simulink model "main_simulation"  (R2023a)
settings: Solver=VariableStepAuto  StartTime=0.0  StopTime=10.0  RelTol=1e-3
values from neighbouring files (symbols this model uses):
  A = [0 1 0 0 0 0 0 0 0 0 0 0 ... (first row only)    [main.m]
  a1 = (Iy - Iz) / Ix    (= 0.245886595932)    [main.m]
  a2 = (Iz - Ix) / Iy    (= -0.245886595932)    [main.m]
  a3 = (Ix - Iy) / Iz    (= 0)    [main.m]
  B = [0 0 0 0 ... (first row only)    [main.m]
  b1 = l / Ix    (= 2894.59486758)    [main.m]
  b2 = l / Iy    (= 2894.59486758)    [main.m]
  b3 = l / Iz    (= 3838.40792639)    [main.m]
  C = [1 0 0 0 0 0 0 0 0 0 0 0 ... (first row only)    [main.m]
  C1 = [0 0 0 0 1 0 0 0 0 0 0 0 ... (first row only)    [main.m]
  D = 0    [main.m]
  F_r = diag([-2,-2,-3,-3,-4,-4,-5,-5])    [main.m]
  g = 9.8    [main.m]
  inv_G_CL_0 = inv(G_CL_0)    [main.m]
  k = place(A, B, [-6.8-7.2i, -6.8+7.2i, -35, -35, -36, -36, -37, -37, -38, -38, -39, -39])    [main.m]
  K_d_LQR = K_LQR(:, 1:12)    [main.m]
  K_place = place(A,B,poles)    [main.m]
  K_q_LQR = K_LQR(:, 13:16)    [main.m]
  L = K'    [main.m]
  L_r = [rand(8,4)]    [main.m]
  m = 0.506    [main.m]
  Q_1 = inv_c_T(:,1:q)    [main.m]
  Q_2 = inv_c_T(:,q+1:n)    [main.m]
  T = lyap(F_r, -A, L_r * C1)    [main.m]
libraries: simulink x2, sim3dlib x1, uavsim3dlib x1
settings Model: Creator=Sheyda  LastModifiedBy=Sheyda

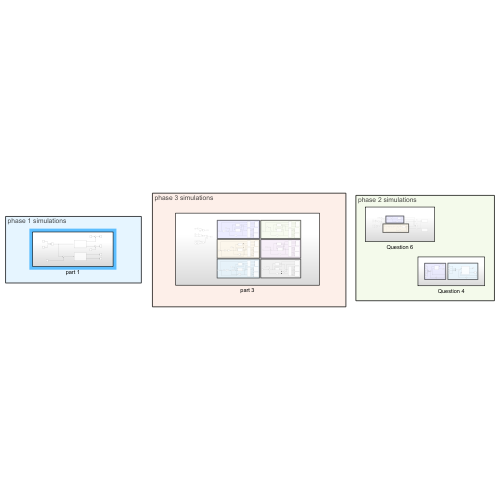
[thumbnail: Simulink's stored preview of the top-level diagram]
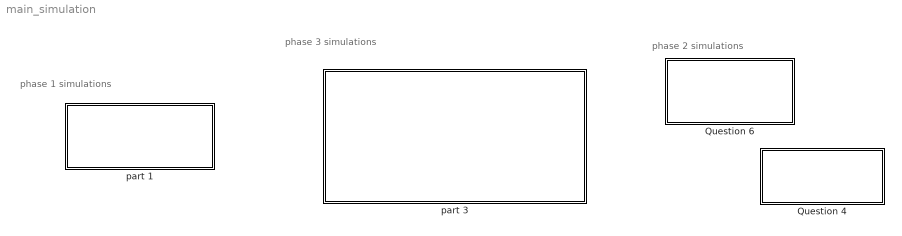
== system main_simulation ==
  note: phase 1 simulations
  note: phase 2 simulations
  note: phase 3 simulations
  Question 4 : Subsystem
  Question 6 : Subsystem
  part 1 : Subsystem
  part 3 : Subsystem

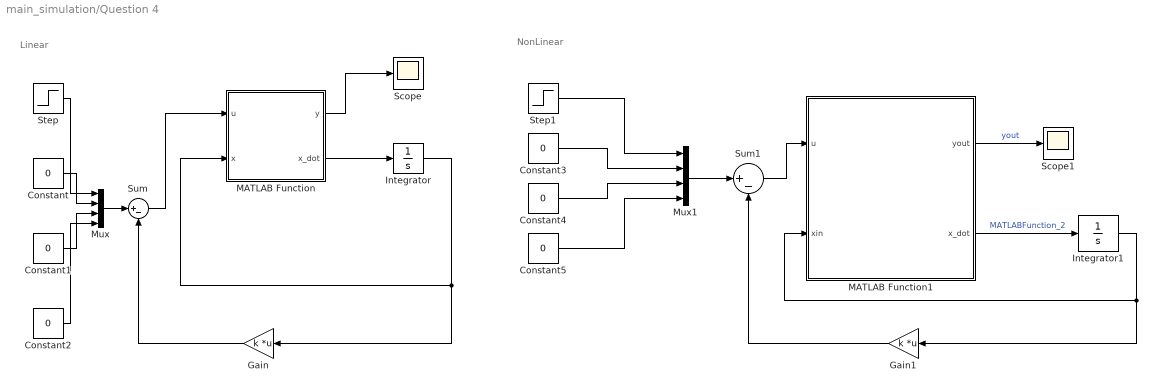
== system main_simulation/Question 4 ==
  note: Linear
  note: NonLinear
  Constant{,1..5} (6 alike) : Constant  Value=0
  Gain : Gain  Gain=k  Multiplication=Matrix(K*u)
  Gain1 : Gain  Gain=k  Multiplication=Matrix(K*u)
  Integrator : Integrator  InitialCondition=[0,0,0,0,0,0,0,0,0,0,0,0]'
  Integrator1 : Integrator  InitialCondition=[0,0,0,0,0,0,0,0,0,0,0,0]'
  MATLAB Function : MATLAB Function  TreatAsAtomicUnit=on
  MATLAB Function1 : MATLAB Function  TreatAsAtomicUnit=on
  Mux : Mux
  Mux1 : Mux
  Scope : Scope
  Scope1 : Scope
  Step : Step  SampleTime=0
  Step1 : Step  SampleTime=0
  Sum : Sum  Inputs=|+-
  Sum1 : Sum  Inputs=|+-
  wires:
  Constant/1 -> Mux/2
  Constant2/1 -> Mux/4
  Constant1/1 -> Mux/3
  Sum/1 -> MATLAB Function/1(u)
  Mux/1 -> Sum/1
  MATLAB Function/2(x_dot) -> Integrator/1
  Gain/1 -> Sum/2
  Integrator/1 -> MATLAB Function/2(x), Gain/1
  Step/1 -> Mux/1
  MATLAB Function/1(y) -> Scope/1
  Constant4/1 -> Mux1/3
  Step1/1 -> Mux1/1
  Constant5/1 -> Mux1/4
  Constant3/1 -> Mux1/2
  Sum1/1 -> MATLAB Function1/1(u)
  MATLAB Function1/2(x_dot) -> Integrator1/1  "MATLABFunction_2"
  MATLAB Function1/1(yout) -> Scope1/1  "yout"
  Mux1/1 -> Sum1/1
  Gain1/1 -> Sum1/2
  Integrator1/1 -> MATLAB Function1/2(xin), Gain1/1

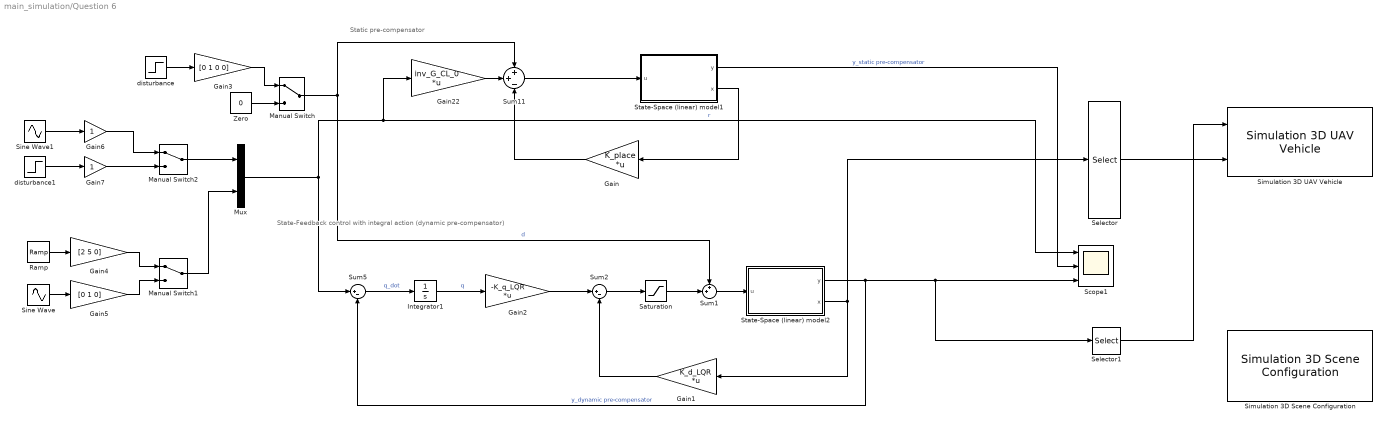
== system main_simulation/Question 6 ==
  note: State-Feedback control with integral action (dynamic pre-compensator)
  note: Static pre-compensator
  Gain : Gain  Gain=K_place  Multiplication=Matrix(K*u)
  Gain1 : Gain  Gain=K_d_LQR  Multiplication=Matrix(K*u)
  Gain2 : Gain  Gain=-K_q_LQR  Multiplication=Matrix(K*u)
  Gain22 : Gain  Gain=inv_G_CL_0  Multiplication=Matrix(K*u)
  Gain3 : Gain  Gain=[0 1 0 0]
  Gain4 : Gain  Gain=[2 5 0]
  Gain5 : Gain  Gain=[0 1 0]
  Gain6 : Gain
  Gain7 : Gain
  Integrator1 : Integrator
  Manual Switch : ManualSwitch
  Manual Switch1 : ManualSwitch
  Manual Switch2 : ManualSwitch
  Mux : Mux  Inputs=2
  Ramp : simulink/Sources/Ramp  slope=1  start=0  InitialOutput=0
  Saturation : Saturate
  Scope1 : Scope  NumInputPorts=3
  Selector : Selector  InputPortWidth=12  IndexOptions=Index vector (dialog)  Indices=[5 3 1]  OutputSizes=1
  Selector1 : Selector  InputPortWidth=4  IndexOptions=Index vector (dialog)  Indices=[3 4 2]  OutputSizes=1
  Simulation 3D Scene Configuration : sim3dlib/Simulation 3D Scene Configuration  Priority=0  ProjectFormat=Default Scenes  SceneDesc=US city block  ProjectName=C:\Program Files\MATLAB\R2023a\toolbox\shared\sim3d_projects\automotive_project\UE4\WindowsNoEditor\VehicleSimulation.exe  ScenePath=/Game/Maps/USCityBlock  EnableOpenDRIVE=off  vehTagList={'Scene Origin'}  vehTag=Scene Origin  OpVisEn=off  Ts=1/60  EnableWindow=on  EnableRemoteAccess=off  EnableWeather=off  SunAltitude=40.0  SunAzimuth=90  clouds=10  wind=1  fog=0  rain=0  EnableGeospatial=off  OriginHeight=200  OriginLatitude=40.744652  OriginLongitude=-73.988864  MapStyle=Aerial  AdditionalAssetIDs=[]  UseAdvancedSunSky=off  SolarTime=11  TimeZone=-5  Day=21  Month=9  Year=2022  UseDaylightSavingTime=on  DSTStartDay=10  DSTStartMonth=3  DSTEndDay=3  DSTEndMonth=11  DSTSwitchHour=2  sensorTag=MainCamera1  sensorId=1  sensorName=MainCamera1  mountLoc=Origin  offsetFlag=off  tmountOffset=[0, 0, 0]  rmountOffset=[0, 0, 0]  HorizontalResolution=1280  VerticalResolution=720  HorizontalFOV=60  mountPoint=[0 0 0]  mountOrientation=[0 0 0]  aMode=4  ID=1  GeoTrigger=Inactive
  Simulation 3D UAV Vehicle : uavsim3dlib/Simulation 3D UAV Vehicle  Priority=-1  Mesh=Quadrotor  MeshPath=/MathWorksUAVContent/UAVs/HexaRotorUAV/HexaRotor.HexaRotor  Color=Black  ActorName=SimulinkVehicle1  UseGlobalFrame=off  InitialTranslation=[0 0 0]  InitialRotation=[0 0 0]  InitialTranslationGlobal=[0 0 0]  InitialGeoOrigin=[0 0 0]  InitialRotationGlobal=[0 0 0]  SampleTime=-1  ActorType=SimulinkVehicle  ID=1  aMode=4  ActorTag=SimulinkVehicle1
  Sine Wave : Sin  SampleTime=0
  Sine Wave1 : Sin  SampleTime=0
  State-Space (linear) model1 : Subsystem
  State-Space (linear) model2 : Subsystem
  Sum1 : Sum  Inputs=++|
  Sum11 : Sum  Inputs=++-
  Sum2 : Sum  Inputs=|+-
  Sum5 : Sum  Inputs=|+-
  Zero : Constant  Value=0
  disturbance : Step  Time=8  After=0.3  SampleTime=0
  disturbance1 : Step  Time=8  After=0.3  SampleTime=0
  wires:
  Gain7/1 -> Manual Switch2/2
  Sum11/1 -> State-Space (linear) model1/1(u)
  Selector/1 -> Simulation 3D UAV Vehicle/2
  Gain6/1 -> Manual Switch2/1
  Saturation/1 -> Sum1/2
  disturbance1/1 -> Gain7/1
  State-Space (linear) model1/2(x) -> Gain/1
  Sine Wave/1 -> Gain5/1
  Sine Wave1/1 -> Gain6/1
  Gain/1 -> Sum11/3
  Manual Switch2/1 -> Mux/1
  Gain4/1 -> Manual Switch1/1
  Selector1/1 -> Simulation 3D UAV Vehicle/1
  Sum2/1 -> Saturation/1
  Gain3/1 -> Manual Switch/1
  State-Space (linear) model2/2(x) -> Selector/1, Gain1/1
  Gain1/1 -> Sum2/2
  Ramp/1 -> Gain4/1
  Manual Switch1/1 -> Mux/2
  State-Space (linear) model2/1(y) -> Sum5/2, Selector1/1, Scope1/3  "y_dynamic pre-compensator"
  Gain5/1 -> Manual Switch1/2
  Gain2/1 -> Sum2/1
  Integrator1/1 -> Gain2/1  "q"
  Zero/1 -> Manual Switch/2
  Mux/1 -> Sum5/1, Scope1/1, Gain22/1  "r"
  Manual Switch/1 -> Sum1/1, Sum11/1  "d"
  Gain22/1 -> Sum11/2
  Sum1/1 -> State-Space (linear) model2/1(u)
  Sum5/1 -> Integrator1/1  "q_dot"
  disturbance/1 -> Gain3/1
  State-Space (linear) model1/1(y) -> Scope1/2  "y_static pre-compensator"

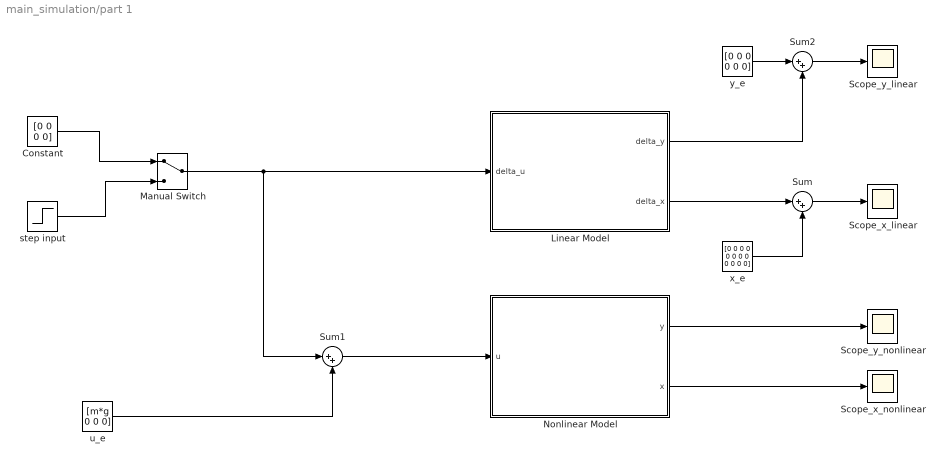
== system main_simulation/part 1 ==
  Constant : Constant  Value=[0 0 0 0]
  Linear Model : Subsystem
  Manual Switch : ManualSwitch
  Nonlinear Model : Subsystem
  Scope_x_linear : Scope
  Scope_x_nonlinear : Scope
  Scope_y_linear : Scope
  Scope_y_nonlinear : Scope
  Sum : Sum  Inputs=|++
  Sum1 : Sum  Inputs=|++
  Sum2 : Sum  Inputs=|++
  step input : Step  After=[100 0 0 0]  SampleTime=0
  u_e : Constant  Value=[m*g 0 0 0]
  x_e : Constant  Value=[0 0 0 0 0 0 0 0 0 0 0 0]
  y_e : Constant  Value=[0 0 0 0 0 0]
  wires:
  y_e/1 -> Sum2/1
  Sum/1 -> Scope_x_linear/1
  Nonlinear Model/2(x) -> Scope_x_nonlinear/1
  Linear Model/1(delta_y) -> Sum2/2
  Linear Model/2(delta_x) -> Sum/1
  Sum2/1 -> Scope_y_linear/1
  x_e/1 -> Sum/2
  Nonlinear Model/1(y) -> Scope_y_nonlinear/1
  u_e/1 -> Sum1/2
  step input/1 -> Manual Switch/2
  Constant/1 -> Manual Switch/1
  Manual Switch/1 -> Linear Model/1(delta_u), Sum1/1
  Sum1/1 -> Nonlinear Model/1(u)

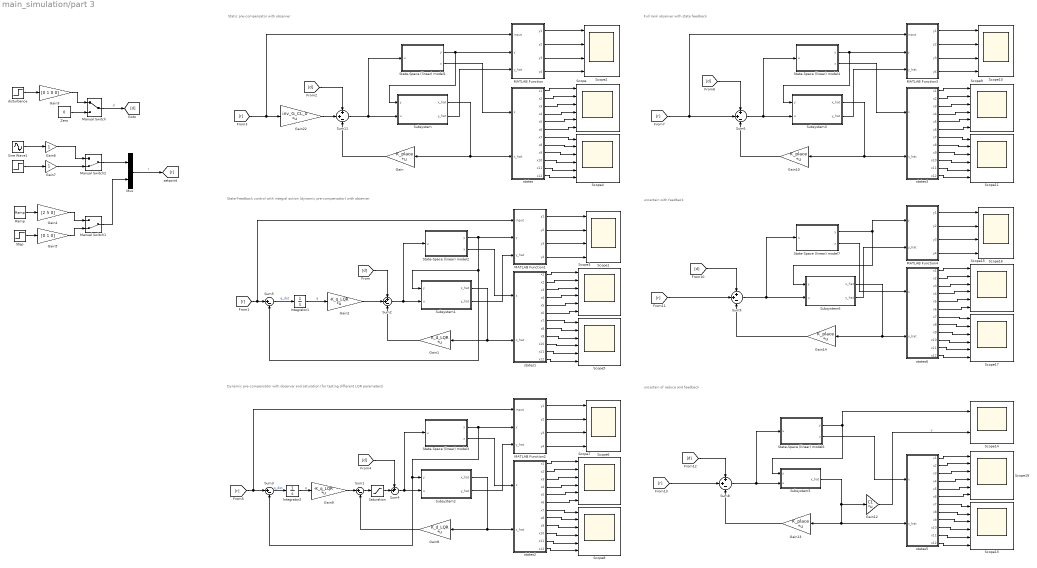
== system main_simulation/part 3 ==
  note: uncertain with feedback
  note: uncertain of reduce and feedback
  note: Full rank observer with state feedback
  note: State-Feedback control with integral action (dynamic pre-compensator) with observer
  note: Dynamic pre-compensator with observer and saturation (for testing different LQR parameters)
  note: Static pre-compensator with observer
  " " : Step  Time=0  After=0.3  SampleTime=0
  Gain{,10,13..14} (4 alike) : Gain  Gain=K_place  Multiplication=Matrix(K*u)
  Gain1 : Gain  Gain=K_d_LQR  Multiplication=Matrix(K*u)
  Gain12 : Gain  Gain=C1  Multiplication=Matrix(K*u)
  Gain2 : Gain  Gain=-K_q_LQR  Multiplication=Matrix(K*u)
  Gain22 : Gain  Gain=inv_G_CL_0  Multiplication=Matrix(K*u)
  Gain3 : Gain  Gain=[0 1 0 0]
  Gain4 : Gain  Gain=[2 5 0]
  Gain5 : Gain  Gain=[0 1 0]
  Gain6 : Gain
  Gain7 : Gain
  Gain8 : Gain  Gain=K_d_LQR  Multiplication=Matrix(K*u)
  Gain9 : Gain  Gain=-K_q_LQR  Multiplication=Matrix(K*u)
  Integrator1 : Integrator
  Integrator2 : Integrator
  MATLAB Function : MATLAB Function  TreatAsAtomicUnit=on
  MATLAB Function1 : MATLAB Function  TreatAsAtomicUnit=on
  MATLAB Function2 : MATLAB Function  TreatAsAtomicUnit=on
  MATLAB Function3 : MATLAB Function  TreatAsAtomicUnit=on
  MATLAB Function4 : MATLAB Function  TreatAsAtomicUnit=on
  Manual Switch : ManualSwitch
  Manual Switch1 : ManualSwitch  CurrentSetting=0
  Manual Switch2 : ManualSwitch  CurrentSetting=0
  Mux : Mux  Inputs=2
  Ramp : simulink/Sources/Ramp  slope=1  start=0  InitialOutput=0
  Saturation : Saturate
  Scope{,3..5,7..9,11,13,15,17,19} (12 alike) : Scope  NumInputPorts=6
  Scope{1..2,6,10,16} (5 alike) : Scope  NumInputPorts=4
  Scope14 : Scope  NumInputPorts=2
  Sine Wave1 : Sin  SampleTime=0
  State-Space (linear) model1 : Subsystem
  State-Space (linear) model2 : Subsystem
  State-Space (linear) model3 : Subsystem
  State-Space (linear) model4 : Subsystem
  State-Space (linear) model6 : Subsystem
  State-Space (linear) model7 : Subsystem
  Step : Step  SampleTime=0
  Subsystem : Subsystem
  Subsystem1 : Subsystem
  Subsystem2 : Subsystem
  Subsystem3 : Subsystem
  Subsystem5 : Subsystem
  Subsystem6 : Subsystem
  Sum1 : Sum  Inputs=|+-
  Sum{2,6,8..9,11} (5 alike) : Sum  Inputs=++-
  Sum3 : Sum  Inputs=|+-
  Sum4 : Sum  Inputs=++|
  Sum5 : Sum  Inputs=|+-
  Zero : Constant  Value=0
  disturbance : Step  Time=8  After=0.3  SampleTime=0
  states : MATLAB Function  TreatAsAtomicUnit=on
  states1 : MATLAB Function  TreatAsAtomicUnit=on
  states2 : MATLAB Function  TreatAsAtomicUnit=on
  states3 : MATLAB Function  TreatAsAtomicUnit=on
  states5 : MATLAB Function  TreatAsAtomicUnit=on
  states6 : MATLAB Function  TreatAsAtomicUnit=on
  wires:
  states5/4(x4) -> Scope19/4
  states5/2(x2) -> Scope19/2
  states5/8(x8) -> Scope13/2
  states5/11(x11) -> Scope13/5
  states5/10(x10) -> Scope13/4
  states5/9(x9) -> Scope13/3
  Sum8/1 -> Subsystem5/2(u), State-Space (linear) model6/1(u)
  Gain13/1 -> Sum8/3
  states6/2(x2) -> Scope15/2
  State-Space (linear) model6/2(x) -> states5/1(x)
  Gain12/1 -> Scope14/2  "y"
  State-Space (linear) model7/2(x) -> states6/1(x)
  states6/9(x9) -> Scope17/3
  State-Space (linear) model7/1(y) -> Subsystem6/1(y), MATLAB Function4/1(y)
  MATLAB Function4/2(y2) -> Scope16/2
  states6/4(x4) -> Scope15/4
  states6/7(x7) -> Scope17/1
  MATLAB Function4/3(y3) -> Scope16/3
  states6/6(x6) -> Scope15/6
  Subsystem6/2(y_hat) -> MATLAB Function4/2(y_hat)
  Subsystem6/1(x_hat) -> states6/2(x_hat), Gain14/1
  states5/7(x7) -> Scope13/1
  states6/12(x12) -> Scope17/6
  states6/8(x8) -> Scope17/2
  [r] -> Sum9/2
  Subsystem5/1(x_hat) -> Gain12/1, states5/2(x_hat), Gain13/1
  Gain14/1 -> Sum9/3
  [r] -> Sum8/2
  [d] -> Sum8/1
  MATLAB Function4/1(y1) -> Scope16/1
  [d] -> Sum9/1
  states6/10(x10) -> Scope17/4
  states2/12(x12) -> Scope8/6
  MATLAB Function3/1(y1) -> Scope10/1
  states2/3(x3) -> Scope7/3
  Sum6/1 -> Subsystem3/2(u), State-Space (linear) model4/1(u)
  states/5(x5) -> Scope/5
  states3/3(x3) -> Scope9/3
  states3/11(x11) -> Scope11/5
  states2/4(x4) -> Scope7/4
  Manual Switch/1 -> [d]  "d"
  Subsystem3/2(y_hat) -> MATLAB Function3/3(y_hat)
  states5/1(x1) -> Scope19/1
  states/4(x4) -> Scope/4
  states3/1(x1) -> Scope9/1
  State-Space (linear) model3/1(y) -> MATLAB Function2/2(y), Subsystem2/1(y), Sum3/2
  [d] -> Sum6/1
  states6/1(x1) -> Scope15/1
  State-Space (linear) model6/1(y) -> Scope14/1, Subsystem5/1(y)
  states3/12(x12) -> Scope11/6
  Gain10/1 -> Sum6/3
  states/2(x2) -> Scope/2
  State-Space (linear) model4/2(x) -> states3/1(x)
  [r] -> Sum5/1, MATLAB Function1/1(input)
  states/6(x6) -> Scope/6
  Sum9/1 -> Subsystem6/2(u), State-Space (linear) model7/1(u)
  states/11(x11) -> Scope4/5
  Gain8/1 -> Sum1/2
  Sine Wave1/1 -> Gain6/1
  MATLAB Function4/4(y4) -> Scope16/4
  MATLAB Function3/3(y3) -> Scope10/3
  Gain1/1 -> Sum2/3
  MATLAB Function1/2(y2) -> Scope1/2
  states6/11(x11) -> Scope17/5
  states3/2(x2) -> Scope9/2
  Sum1/1 -> Saturation/1
  states3/8(x8) -> Scope11/2
  [d] -> Sum4/1
  MATLAB Function3/2(y2) -> Scope10/2
  MATLAB Function2/2(y2) -> Scope6/2
  states1/3(x3) -> Scope3/3
  Gain2/1 -> Sum2/2
  MATLAB Function2/1(y1) -> Scope6/1
  states3/4(x4) -> Scope9/4
  MATLAB Function3/4(y4) -> Scope10/4
  State-Space (linear) model4/1(y) -> Subsystem3/1(y), MATLAB Function3/2(y)
  states/7(x7) -> Scope4/1
  states2/8(x8) -> Scope8/2
  Subsystem1/2(y_hat) -> MATLAB Function1/3(y_hat)
  Subsystem3/1(x_hat) -> states3/2(x_hat), Gain10/1
  states5/6(x6) -> Scope19/6
  Gain22/1 -> Sum11/2
  State-Space (linear) model3/2(x) -> states2/1(x)
  states3/10(x10) -> Scope11/4
  states1/11(x11) -> Scope5/5
  states1/5(x5) -> Scope3/5
  states1/10(x10) -> Scope5/4
  states1/2(x2) -> Scope3/2
  states2/11(x11) -> Scope8/5
  states2/5(x5) -> Scope7/5
  states3/7(x7) -> Scope11/1
  [r] -> Sum6/2, MATLAB Function3/1(input)
  Sum4/1 -> State-Space (linear) model3/1(u), Subsystem2/2(u)
  states3/9(x9) -> Scope11/3
  states1/6(x6) -> Scope3/6
  states2/10(x10) -> Scope8/4
  states2/7(x7) -> Scope8/1
  Subsystem2/1(x_hat) -> Gain8/1, states2/2(x_hat)
  states2/2(x2) -> Scope7/2
  [r] -> Sum3/1, MATLAB Function2/1(input)
  Integrator1/1 -> Gain2/1  "q"
  states/12(x12) -> Scope4/6
  states3/6(x6) -> Scope9/6
  Gain9/1 -> Sum1/1
  states5/3(x3) -> Scope19/3
  Saturation/1 -> Sum4/2
  Sum5/1 -> Integrator1/1  "q_dot"
  states1/8(x8) -> Scope5/2
  states/10(x10) -> Scope4/4
  Subsystem2/2(y_hat) -> MATLAB Function2/3(y_hat)
  states2/1(x1) -> Scope7/1
  [d] -> Sum2/1
  states5/5(x5) -> Scope19/5
  Sum3/1 -> Integrator2/1  "q_dot"
  MATLAB Function1/4(y4) -> Scope1/4
  Integrator2/1 -> Gain9/1  "q"
  State-Space (linear) model2/1(y) -> MATLAB Function1/2(y), Subsystem1/1(y), Sum5/2
  MATLAB Function2/4(y4) -> Scope6/4
  states1/7(x7) -> Scope5/1
  states6/5(x5) -> Scope15/5
  MATLAB Function/1(y1) -> Scope2/1
  Gain4/1 -> Manual Switch1/1
  MATLAB Function/2(y2) -> Scope2/2
  State-Space (linear) model2/2(x) -> states1/1(x)
  states2/9(x9) -> Scope8/3
  states6/3(x3) -> Scope15/3
  states1/9(x9) -> Scope5/3
  State-Space (linear) model1/2(x) -> states/1(x)
  MATLAB Function1/3(y3) -> Scope1/3
  states1/12(x12) -> Scope5/6
  states2/6(x6) -> Scope7/6
  states1/4(x4) -> Scope3/4
  State-Space (linear) model1/1(y) -> Subsystem/1(y), MATLAB Function/2(y)
  states/8(x8) -> Scope4/2
  MATLAB Function/3(y3) -> Scope2/3
  Sum2/1 -> Subsystem1/2(u), State-Space (linear) model2/1(u)
  MATLAB Function/4(y4) -> Scope2/4
  Subsystem/2(y_hat) -> MATLAB Function/3(y_hat)
  MATLAB Function1/1(y1) -> Scope1/1
  MATLAB Function2/3(y3) -> Scope6/3
  Sum11/1 -> State-Space (linear) model1/1(u), Subsystem/2(u)
  states/3(x3) -> Scope/3
  Gain7/1 -> Manual Switch2/2
  Gain/1 -> Sum11/3
  states3/5(x5) -> Scope9/5
  states5/12(x12) -> Scope13/6
  Subsystem/1(x_hat) -> states/2(x_hat), Gain/1
  states/1(x1) -> Scope/1
  disturbance/1 -> Gain3/1
  states1/1(x1) -> Scope3/1
  Ramp/1 -> Gain4/1
  [d] -> Sum11/1
  [r] -> MATLAB Function/1(input), Gain22/1
  Subsystem1/1(x_hat) -> Gain1/1, states1/2(x_hat)
  Manual Switch1/1 -> Mux/2
  Mux/1 -> [r]  "r"
  Zero/1 -> Manual Switch/2
  Gain6/1 -> Manual Switch2/1
  Gain5/1 -> Manual Switch1/2
  states/9(x9) -> Scope4/3
  Step/1 -> Gain5/1
  Manual Switch2/1 -> Mux/1
  " "/1 -> Gain7/1
  Gain3/1 -> Manual Switch/1

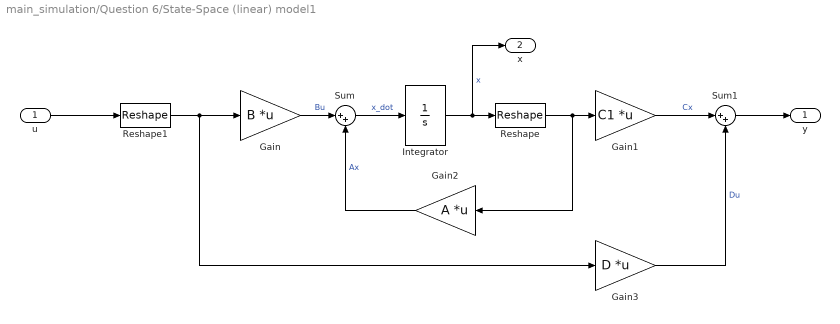
== system main_simulation/Question 6/State-Space (linear) model1 ==
  u : Inport
  Gain : Gain  Gain=B  Multiplication=Matrix(K*u)
  Gain1 : Gain  Gain=C1  Multiplication=Matrix(K*u)
  Gain2 : Gain  Gain=A  Multiplication=Matrix(K*u)
  Gain3 : Gain  Gain=D  Multiplication=Matrix(K*u)
  Integrator : Integrator  InitialCondition=[0; 0; 0; 0; 0; 0; 0; 0; 0; 0; 0; 0]
  Reshape : Reshape  OutputDimensionality=Column vector (2-D)  OutputDimensions=[12,1]
  Reshape1 : Reshape  OutputDimensionality=Column vector (2-D)
  Sum : Sum  Inputs=|++
  Sum1 : Sum  Inputs=|++
  y : Outport
  x : Outport  Port=2
  wires:
  Gain/1 -> Sum/1  "Bu"
  Sum/1 -> Integrator/1  "x_dot"
  Integrator/1 -> x/1, Reshape/1  "x"
  Gain2/1 -> Sum/2  "Ax"
  Reshape/1 -> Gain2/1, Gain1/1
  Reshape1/1 -> Gain/1, Gain3/1
  u/1 -> Reshape1/1
  Gain3/1 -> Sum1/2  "Du"
  Gain1/1 -> Sum1/1  "Cx"
  Sum1/1 -> y/1

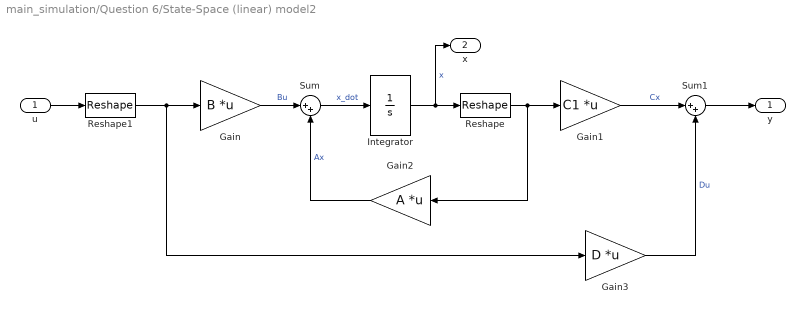
== system main_simulation/Question 6/State-Space (linear) model2 ==
  u : Inport
  Gain : Gain  Gain=B  Multiplication=Matrix(K*u)
  Gain1 : Gain  Gain=C1  Multiplication=Matrix(K*u)
  Gain2 : Gain  Gain=A  Multiplication=Matrix(K*u)
  Gain3 : Gain  Gain=D  Multiplication=Matrix(K*u)
  Integrator : Integrator  InitialCondition=[0; 0; 0; 0; 0; 0; 0; 0; 0; 0; 0; 0]
  Reshape : Reshape  OutputDimensionality=Column vector (2-D)  OutputDimensions=[12,1]
  Reshape1 : Reshape  OutputDimensionality=Column vector (2-D)
  Sum : Sum  Inputs=|++
  Sum1 : Sum  Inputs=|++
  y : Outport
  x : Outport  Port=2
  wires:
  Gain/1 -> Sum/1  "Bu"
  Sum/1 -> Integrator/1  "x_dot"
  Integrator/1 -> x/1, Reshape/1  "x"
  Gain1/1 -> Sum1/1  "Cx"
  Gain2/1 -> Sum/2  "Ax"
  Reshape/1 -> Gain2/1, Gain1/1
  Reshape1/1 -> Gain3/1, Gain/1
  u/1 -> Reshape1/1
  Sum1/1 -> y/1
  Gain3/1 -> Sum1/2  "Du"

== system main_simulation/part 1/Linear Model ==
  delta_u : Inport
  Integrator : Integrator  InitialCondition=[0,0.1,0,0,0,0,0,0,0,0,0,0].'  WrapState=on  WrappedStateUpperValue=[pi; inf; pi; inf; pi; inf; inf; inf; inf; inf; inf; inf]  WrappedStateLowerValue=[-pi; -inf; -pi; -inf; -pi; -inf; -inf; -inf; -inf; -inf; -inf; -inf]
  MATLAB Function : MATLAB Function  TreatAsAtomicUnit=on
  SS block : Subsystem
  Scope : Scope  NumInputPorts=2
  Scope1 : Scope
  Scope2 : Scope
  delta_y : Outport
  delta_x : Outport  Port=2
  wires:
  MATLAB Function/2(x_dot) -> Integrator/1
  Integrator/1 -> delta_x/1, Scope2/1, MATLAB Function/2(X)  "x"
  delta_u/1 -> MATLAB Function/1(u), SS block/1(u)
  MATLAB Function/1(y) -> delta_y/1, Scope/2
  SS block/1(y) -> Scope/1
  SS block/2(x) -> Scope1/1

== system main_simulation/part 1/Nonlinear Model ==
  u : Inport
  Integrator : Integrator  InitialCondition=[0,0.1,0,0,0,0,0,0,0,0,0,0].'  WrapState=on  WrappedStateUpperValue=[pi; inf; pi; inf; pi; inf; inf; inf; inf; inf; inf; inf]  WrappedStateLowerValue=[-pi; -inf; -pi; -inf; -pi; -inf; -inf; -inf; -inf; -inf; -inf; -inf]
  MATLAB Function : MATLAB Function  TreatAsAtomicUnit=on
  y : Outport
  x : Outport  Port=2
  wires:
  MATLAB Function/2(X_dot) -> Integrator/1
  Integrator/1 -> x/1, MATLAB Function/2(X)
  u/1 -> MATLAB Function/1(U)
  MATLAB Function/1(y) -> y/1

== system main_simulation/part 3/State-Space (linear) model1 ==
  u : Inport
  Gain : Gain  Gain=B  Multiplication=Matrix(K*u)
  Gain1 : Gain  Gain=C1  Multiplication=Matrix(K*u)
  Gain2 : Gain  Gain=A  Multiplication=Matrix(K*u)
  Gain3 : Gain  Gain=D  Multiplication=Matrix(K*u)
  Integrator : Integrator  InitialCondition=[0; 0; 0; 0; 0; 0; 0; 0; 0; 0; 0; 0]
  Reshape : Reshape  OutputDimensionality=Column vector (2-D)  OutputDimensions=[12,1]
  Reshape1 : Reshape  OutputDimensionality=Column vector (2-D)
  Sum : Sum  Inputs=|++
  Sum1 : Sum  Inputs=|++
  y : Outport
  x : Outport  Port=2
  wires:
  Gain/1 -> Sum/1  "Bu"
  Sum/1 -> Integrator/1  "x_dot"
  Integrator/1 -> x/1, Reshape/1  "x"
  Gain2/1 -> Sum/2  "Ax"
  Reshape/1 -> Gain2/1, Gain1/1
  Reshape1/1 -> Gain/1, Gain3/1
  u/1 -> Reshape1/1
  Gain3/1 -> Sum1/2  "Du"
  Gain1/1 -> Sum1/1  "Cx"
  Sum1/1 -> y/1

== system main_simulation/part 3/State-Space (linear) model2 ==
  u : Inport
  Gain : Gain  Gain=B  Multiplication=Matrix(K*u)
  Gain1 : Gain  Gain=C1  Multiplication=Matrix(K*u)
  Gain2 : Gain  Gain=A  Multiplication=Matrix(K*u)
  Gain3 : Gain  Gain=D  Multiplication=Matrix(K*u)
  Integrator : Integrator  InitialCondition=[0; 0; 0; 0; 0; 0; 0; 0; 0; 0; 0; 0]
  Reshape : Reshape  OutputDimensionality=Column vector (2-D)  OutputDimensions=[12,1]
  Reshape1 : Reshape  OutputDimensionality=Column vector (2-D)
  Sum : Sum  Inputs=|++
  Sum1 : Sum  Inputs=|++
  y : Outport
  x : Outport  Port=2
  wires:
  Gain/1 -> Sum/1  "Bu"
  Sum/1 -> Integrator/1  "x_dot"
  Integrator/1 -> x/1, Reshape/1  "x"
  Gain1/1 -> Sum1/1  "Cx"
  Gain2/1 -> Sum/2  "Ax"
  Reshape/1 -> Gain2/1, Gain1/1
  Reshape1/1 -> Gain3/1, Gain/1
  u/1 -> Reshape1/1
  Sum1/1 -> y/1
  Gain3/1 -> Sum1/2  "Du"

== system main_simulation/part 3/State-Space (linear) model3 ==
  u : Inport
  Gain : Gain  Gain=B  Multiplication=Matrix(K*u)
  Gain1 : Gain  Gain=C1  Multiplication=Matrix(K*u)
  Gain2 : Gain  Gain=A  Multiplication=Matrix(K*u)
  Gain3 : Gain  Gain=D  Multiplication=Matrix(K*u)
  Integrator : Integrator  InitialCondition=[0; 0; 0; 0; 0; 0; 0; 0; 0; 0; 0; 0]
  Reshape : Reshape  OutputDimensionality=Column vector (2-D)  OutputDimensions=[12,1]
  Reshape1 : Reshape  OutputDimensionality=Column vector (2-D)
  Sum : Sum  Inputs=|++
  Sum1 : Sum  Inputs=|++
  y : Outport
  x : Outport  Port=2
  wires:
  Gain/1 -> Sum/1  "Bu"
  Sum/1 -> Integrator/1  "x_dot"
  Integrator/1 -> x/1, Reshape/1  "x"
  Gain1/1 -> Sum1/1  "Cx"
  Gain2/1 -> Sum/2  "Ax"
  Reshape/1 -> Gain2/1, Gain1/1
  Reshape1/1 -> Gain3/1, Gain/1
  u/1 -> Reshape1/1
  Sum1/1 -> y/1
  Gain3/1 -> Sum1/2  "Du"

== system main_simulation/part 3/State-Space (linear) model4 ==
  u : Inport
  Gain : Gain  Gain=B  Multiplication=Matrix(K*u)
  Gain1 : Gain  Gain=C1  Multiplication=Matrix(K*u)
  Gain2 : Gain  Gain=A  Multiplication=Matrix(K*u)
  Gain3 : Gain  Gain=D  Multiplication=Matrix(K*u)
  Integrator : Integrator  InitialCondition=[0; 0; 0; 0; 0; 0; 0; 0; 0; 0; 0; 0]
  Reshape : Reshape  OutputDimensionality=Column vector (2-D)  OutputDimensions=[12,1]
  Reshape1 : Reshape  OutputDimensionality=Column vector (2-D)
  Sum : Sum  Inputs=|++
  Sum1 : Sum  Inputs=|++
  y : Outport
  x : Outport  Port=2
  wires:
  Gain/1 -> Sum/1  "Bu"
  Sum/1 -> Integrator/1  "x_dot"
  Integrator/1 -> x/1, Reshape/1  "x"
  Gain2/1 -> Sum/2  "Ax"
  Reshape/1 -> Gain2/1, Gain1/1
  Reshape1/1 -> Gain/1, Gain3/1
  u/1 -> Reshape1/1
  Gain3/1 -> Sum1/2  "Du"
  Gain1/1 -> Sum1/1  "Cx"
  Sum1/1 -> y/1

== system main_simulation/part 3/State-Space (linear) model6 ==
  u : Inport
  Gain : Gain  Gain=B  Multiplication=Matrix(K*u)
  Gain1 : Gain  Gain=C1  Multiplication=Matrix(K*u)
  Gain2 : Gain  Gain=A*1.2  Multiplication=Matrix(K*u)
  Gain3 : Gain  Gain=D  Multiplication=Matrix(K*u)
  Integrator : Integrator  InitialCondition=[0; 0; 0; 0; 0; 0; 0; 0; 0; 0; 0; 0]
  Reshape : Reshape  OutputDimensionality=Column vector (2-D)  OutputDimensions=[12,1]
  Reshape1 : Reshape  OutputDimensionality=Column vector (2-D)
  Sum : Sum  Inputs=|++
  Sum1 : Sum  Inputs=|++
  y : Outport
  x : Outport  Port=2
  wires:
  Gain/1 -> Sum/1  "Bu"
  Sum/1 -> Integrator/1  "x_dot"
  Integrator/1 -> x/1, Reshape/1  "x"
  Gain2/1 -> Sum/2  "Ax"
  Reshape/1 -> Gain2/1, Gain1/1
  Reshape1/1 -> Gain/1, Gain3/1
  u/1 -> Reshape1/1
  Gain3/1 -> Sum1/2  "Du"
  Gain1/1 -> Sum1/1  "Cx"
  Sum1/1 -> y/1

== system main_simulation/part 3/State-Space (linear) model7 ==
  u : Inport
  Gain : Gain  Gain=B  Multiplication=Matrix(K*u)
  Gain1 : Gain  Gain=C1  Multiplication=Matrix(K*u)
  Gain2 : Gain  Gain=A*1.2  Multiplication=Matrix(K*u)
  Gain3 : Gain  Gain=D  Multiplication=Matrix(K*u)
  Integrator : Integrator
  Reshape : Reshape  OutputDimensionality=Column vector (2-D)  OutputDimensions=[12,1]
  Reshape1 : Reshape  OutputDimensionality=Column vector (2-D)
  Sum : Sum  Inputs=|++
  Sum1 : Sum  Inputs=|++
  y : Outport
  x : Outport  Port=2
  wires:
  Gain/1 -> Sum/1  "Bu"
  Sum/1 -> Integrator/1  "x_dot"
  Integrator/1 -> x/1, Reshape/1  "x"
  Gain2/1 -> Sum/2  "Ax"
  Reshape/1 -> Gain2/1, Gain1/1
  Reshape1/1 -> Gain/1, Gain3/1
  u/1 -> Reshape1/1
  Gain3/1 -> Sum1/2  "Du"
  Gain1/1 -> Sum1/1  "Cx"
  Sum1/1 -> y/1

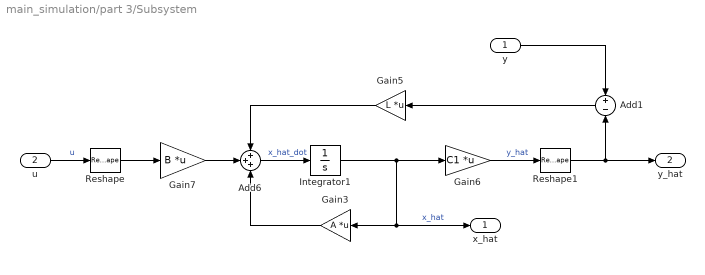
== system main_simulation/part 3/Subsystem ==
  y : Inport
  u : Inport  Port=2
  Add1 : Sum  Inputs=+-
  Add6 : Sum  Inputs=+++
  Gain3 : Gain  Gain=A  Multiplication=Matrix(K*u)
  Gain5 : Gain  Gain=L  Multiplication=Matrix(K*u)
  Gain6 : Gain  Gain=C1  Multiplication=Matrix(K*u)
  Gain7 : Gain  Gain=B  Multiplication=Matrix(K*u)
  Integrator1 : Integrator
  Reshape : Reshape  OutputDimensionality=Column vector (2-D)
  Reshape1 : Reshape  OutputDimensionality=Column vector (2-D)
  x_hat : Outport
  y_hat : Outport  Port=2
  wires:
  Gain3/1 -> Add6/3
  Integrator1/1 -> Gain6/1, x_hat/1, Gain3/1  "x_hat"
  u/1 -> Reshape/1  "u"
  Gain6/1 -> Reshape1/1  "y_hat"
  Gain7/1 -> Add6/2
  Gain5/1 -> Add6/1
  y/1 -> Add1/1
  Add6/1 -> Integrator1/1  "x_hat_dot"
  Add1/1 -> Gain5/1
  Reshape/1 -> Gain7/1
  Reshape1/1 -> y_hat/1, Add1/2

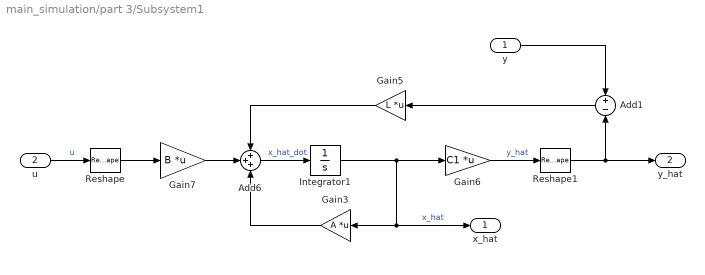
== system main_simulation/part 3/Subsystem1 ==
  y : Inport
  u : Inport  Port=2
  Add1 : Sum  Inputs=+-
  Add6 : Sum  Inputs=+++
  Gain3 : Gain  Gain=A  Multiplication=Matrix(K*u)
  Gain5 : Gain  Gain=L  Multiplication=Matrix(K*u)
  Gain6 : Gain  Gain=C1  Multiplication=Matrix(K*u)
  Gain7 : Gain  Gain=B  Multiplication=Matrix(K*u)
  Integrator1 : Integrator
  Reshape : Reshape  OutputDimensionality=Column vector (2-D)
  Reshape1 : Reshape  OutputDimensionality=Column vector (2-D)
  x_hat : Outport
  y_hat : Outport  Port=2
  wires:
  Reshape1/1 -> y_hat/1, Add1/2
  Gain7/1 -> Add6/2
  Add6/1 -> Integrator1/1  "x_hat_dot"
  Add1/1 -> Gain5/1
  y/1 -> Add1/1
  u/1 -> Reshape/1  "u"
  Gain6/1 -> Reshape1/1  "y_hat"
  Reshape/1 -> Gain7/1
  Gain3/1 -> Add6/3
  Gain5/1 -> Add6/1
  Integrator1/1 -> Gain6/1, x_hat/1, Gain3/1  "x_hat"

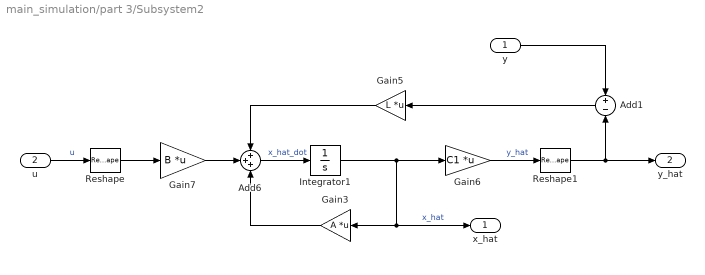
== system main_simulation/part 3/Subsystem2 ==
  y : Inport
  u : Inport  Port=2
  Add1 : Sum  Inputs=+-
  Add6 : Sum  Inputs=+++
  Gain3 : Gain  Gain=A  Multiplication=Matrix(K*u)
  Gain5 : Gain  Gain=L  Multiplication=Matrix(K*u)
  Gain6 : Gain  Gain=C1  Multiplication=Matrix(K*u)
  Gain7 : Gain  Gain=B  Multiplication=Matrix(K*u)
  Integrator1 : Integrator
  Reshape : Reshape  OutputDimensionality=Column vector (2-D)
  Reshape1 : Reshape  OutputDimensionality=Column vector (2-D)
  x_hat : Outport
  y_hat : Outport  Port=2
  wires:
  Reshape1/1 -> y_hat/1, Add1/2
  Gain7/1 -> Add6/2
  Add6/1 -> Integrator1/1  "x_hat_dot"
  Add1/1 -> Gain5/1
  y/1 -> Add1/1
  u/1 -> Reshape/1  "u"
  Gain6/1 -> Reshape1/1  "y_hat"
  Reshape/1 -> Gain7/1
  Gain3/1 -> Add6/3
  Gain5/1 -> Add6/1
  Integrator1/1 -> Gain6/1, x_hat/1, Gain3/1  "x_hat"

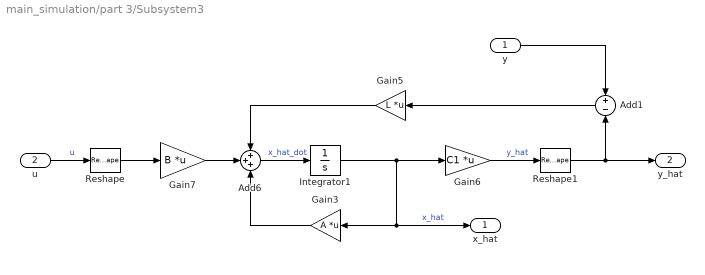
== system main_simulation/part 3/Subsystem3 ==
  y : Inport
  u : Inport  Port=2
  Add1 : Sum  Inputs=+-
  Add6 : Sum  Inputs=+++
  Gain3 : Gain  Gain=A  Multiplication=Matrix(K*u)
  Gain5 : Gain  Gain=L  Multiplication=Matrix(K*u)
  Gain6 : Gain  Gain=C1  Multiplication=Matrix(K*u)
  Gain7 : Gain  Gain=B  Multiplication=Matrix(K*u)
  Integrator1 : Integrator
  Reshape : Reshape  OutputDimensionality=Column vector (2-D)
  Reshape1 : Reshape  OutputDimensionality=Column vector (2-D)
  x_hat : Outport
  y_hat : Outport  Port=2
  wires:
  Gain3/1 -> Add6/3
  Integrator1/1 -> Gain6/1, x_hat/1, Gain3/1  "x_hat"
  u/1 -> Reshape/1  "u"
  Gain6/1 -> Reshape1/1  "y_hat"
  Gain7/1 -> Add6/2
  Gain5/1 -> Add6/1
  y/1 -> Add1/1
  Add6/1 -> Integrator1/1  "x_hat_dot"
  Add1/1 -> Gain5/1
  Reshape/1 -> Gain7/1
  Reshape1/1 -> y_hat/1, Add1/2

== system main_simulation/part 3/Subsystem5 ==
  y : Inport
  u : Inport  Port=2
  Gain10 : Gain  Gain=T * B  Multiplication=Matrix(K*u)
  Gain11 : Gain  Gain=F_r  Multiplication=Matrix(K*u)
  Gain12 : Gain  Gain=L_r  Multiplication=Matrix(K*u)
  Gain13 : Gain  Gain=Q_2  Multiplication=Matrix(K*u)
  Gain14 : Gain  Gain=Q_1  Multiplication=Matrix(K*u)
  Integrator : Integrator
  Sum : Sum  Inputs=+++
  Sum3 : Sum  Inputs=|++
  x_hat : Outport
  wires:
  Gain13/1 -> Sum3/1  "Q2z"
  y/1 -> Gain12/1, Gain14/1  "y"
  Sum/1 -> Integrator/1  "z_dot"
  Sum3/1 -> x_hat/1  "x_hat"
  Gain14/1 -> Sum3/2  "Q1y"
  u/1 -> Gain10/1
  Gain12/1 -> Sum/2  "Ly"
  Gain10/1 -> Sum/1  "TBu"
  Integrator/1 -> Gain13/1, Gain11/1  "z"
  Gain11/1 -> Sum/3  "Fz"

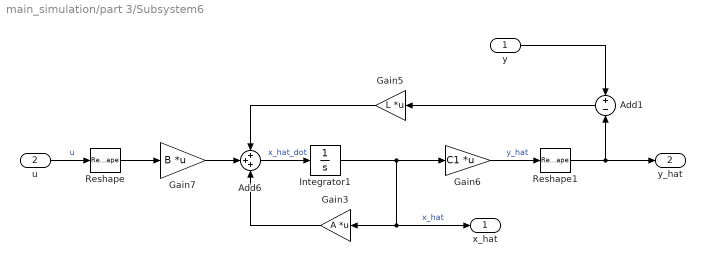
== system main_simulation/part 3/Subsystem6 ==
  y : Inport
  u : Inport  Port=2
  Add1 : Sum  Inputs=+-
  Add6 : Sum  Inputs=+++
  Gain3 : Gain  Gain=A  Multiplication=Matrix(K*u)
  Gain5 : Gain  Gain=L  Multiplication=Matrix(K*u)
  Gain6 : Gain  Gain=C1  Multiplication=Matrix(K*u)
  Gain7 : Gain  Gain=B  Multiplication=Matrix(K*u)
  Integrator1 : Integrator
  Reshape : Reshape  OutputDimensionality=Column vector (2-D)
  Reshape1 : Reshape  OutputDimensionality=Column vector (2-D)
  x_hat : Outport
  y_hat : Outport  Port=2
  wires:
  Gain3/1 -> Add6/3
  Integrator1/1 -> Gain6/1, x_hat/1, Gain3/1  "x_hat"
  u/1 -> Reshape/1  "u"
  Gain6/1 -> Reshape1/1  "y_hat"
  Gain7/1 -> Add6/2
  Gain5/1 -> Add6/1
  y/1 -> Add1/1
  Add6/1 -> Integrator1/1  "x_hat_dot"
  Add1/1 -> Gain5/1
  Reshape/1 -> Gain7/1
  Reshape1/1 -> y_hat/1, Add1/2

== system main_simulation/part 1/Linear Model/SS block ==
  u : Inport
  Gain : Gain  Gain=B  Multiplication=Matrix(K*u)
  Gain1 : Gain  Gain=A  Multiplication=Matrix(K*u)
  Gain3 : Gain  Gain=C  Multiplication=Matrix(K*u)
  Integrator : Integrator  InitialCondition=[0,0.1,0,0,0,0,0,0,0,0,0,0].'  WrapState=on  WrappedStateUpperValue=[pi; inf; pi; inf; pi; inf; inf; inf; inf; inf; inf; inf]  WrappedStateLowerValue=[-pi; -inf; -pi; -inf; -pi; -inf; -inf; -inf; -inf; -inf; -inf; -inf]
  Reshape : Reshape  OutputDimensionality=Column vector (2-D)
  Reshape1 : Reshape  OutputDimensionality=Column vector (2-D)
  Sum : Sum  Inputs=|++
  y : Outport
  x : Outport  Port=2
  wires:
  Sum/1 -> Integrator/1  "x_dot"
  Reshape/1 -> Gain/1
  Integrator/1 -> Reshape1/1, x/1  "x"
  u/1 -> Reshape/1
  Gain/1 -> Sum/1  "Bu"
  Gain3/1 -> y/1  "Cx"
  Reshape1/1 -> Gain1/1, Gain3/1
  Gain1/1 -> Sum/2  "Ax"

== matlab function main_simulation/part 3/MATLAB Function3 ==
  data: input input; y input; y1 output; y_hat input; y2 output; y3 output; y4 output
function [y1 ,y2 ,y3 ,y4]  = CP(input, y, y_hat)

 y1=[input(1), y(1), y_hat(1)];
 y2=[input(2), y(2), y_hat(2)];
 y3=[input(3), y(3), y_hat(3)];
 y4=[input(4), y(4), y_hat(4)];

== matlab function main_simulation/part 3/states3 ==
  data: x input; x1 output; x_hat input; x2 output; x3 output; x4 output; x5 output; x6 output; x7 output; x8 output; x9 output; x10 output; x11 output; x12 output
function [x1 ,x2, x3, x4, x5, x6, x7, x8, x9, x10, x11, x12]  = CP(x, x_hat)

 x1=[x(1), x_hat(1)];
 x2=[x(2), x_hat(2)];
 x3=[x(3), x_hat(3)];
 x4=[x(4), x_hat(4)];
 x5=[x(5), x_hat(5)];
 x6=[x(6), x_hat(6)];
 x7=[x(7), x_hat(7)];
 x8=[x(8), x_hat(8)];
 x9=[x(9), x_hat(9)];
 x10=[x(10), x_hat(10)];
 x11=[x(11), x_hat(11)];
 x12=[x(12), x_hat(12)];

== matlab function main_simulation/part 3/MATLAB Function4 ==
  data: y input; y1 output; y_hat input; y2 output; y3 output; y4 output
function [y1 ,y2 ,y3 ,y4]  = CP(y, y_hat)

 y1=[y(1), y_hat(1)];
 y2=[y(2), y_hat(2)];
 y3=[y(3), y_hat(3)];
 y4=[y(4), y_hat(4)];

== matlab function main_simulation/Question 4/MATLAB Function ==
  data: u input; y output; x input; x_dot output
function [y,x_dot] = fcn(u,x)
L  = 0.235 %m
Ix = 8.11858 * 10^(-5) % kg m2
Iy = 8.11858 * 10^(-5) % kg m2
Iz = 6.12233 * 10^(-5) % kg m2
b1 = L/Ix
b2 = L/Iy
b3 = L/Iz
m  = 0.506 % kg
g  = 9.8   % m s2
B = [0 0 0 0;
     0 b1 0 0; 
     0 0 0 0; 
     0 0 b2 0; 
     0 0 0 0; 
     0 0 0 b3; 
     0 0 0 0; 
     (1/m) 0 0 0; 
     0 0 0 0; 
     0 0 0 0;
     0 0 0 0;
     0 0 0 0];
A = [0 1 0 0 0 0 0 0 0 0 0 0 ;
     0 0 0 0 0 0 0 0 0 0 0 0;
     0 0 0 1 0 0 0 0 0 0 0 0;
     0 0 0 0 0 0 0 0 0 0 0 0;
     0 0 0 0 0 1 0 0 0 0 0 0;
     0 0 0 0 0 0 0 0 0 0 0 0;
     0 0 0 0 0 0 0 1 0 0 0 0;
     0 0 0 0 0 0 0 0 0 0 0 0;
     0 0 0 0 0 0 0 0 0 1 0 0;
     0 0 g 0 0 0 0 0 0 0 0 0;
     0 0 0 0 0 0 0 0 0 0 0 1;
     -g 0 0 0 0 0 0 0 0 0 0 0];

c = [1 0 0 0 0 0 0 0 0 0 0 0;
0 0 1 0 0 0 0 0 0 0 0 0;
0 0 0 0 1 0 0 0 0 0 0 0;
0 0 0 0 0 0 1 0 0 0 0 0;
0 0 0 0 0 0 0 0 1 0 0 0;
0 0 0 0 0 0 0 0 0 0 1 0];
 
D = [0,0,0,0;
    0,0,0,0;
    0,0,0,0;
    0,0,0,0;
    0,0,0,0;
    0,0,0,0]; 

x_dot = A*x + B*u;

y = c*x + D*u;

== matlab function main_simulation/part 3/states5 ==
  data: x input; x1 output; x_hat input; x2 output; x3 output; x4 output; x5 output; x6 output; x7 output; x8 output; x9 output; x10 output; x11 output; x12 output
function [x1 ,x2, x3, x4, x5, x6, x7, x8, x9, x10, x11, x12]  = CP(x, x_hat)

 x1=[x(1), x_hat(1)];
 x2=[x(2), x_hat(2)];
 x3=[x(3), x_hat(3)];
 x4=[x(4), x_hat(4)];
 x5=[x(5), x_hat(5)];
 x6=[x(6), x_hat(6)];
 x7=[x(7), x_hat(7)];
 x8=[x(8), x_hat(8)];
 x9=[x(9), x_hat(9)];
 x10=[x(10), x_hat(10)];
 x11=[x(11), x_hat(11)];
 x12=[x(12), x_hat(12)];

== matlab function main_simulation/part 3/states6 ==
  data: x input; x1 output; x_hat input; x2 output; x3 output; x4 output; x5 output; x6 output; x7 output; x8 output; x9 output; x10 output; x11 output; x12 output
function [x1 ,x2, x3, x4, x5, x6, x7, x8, x9, x10, x11, x12]  = CP(x, x_hat)

 x1=[x(1), x_hat(1)];
 x2=[x(2), x_hat(2)];
 x3=[x(3), x_hat(3)];
 x4=[x(4), x_hat(4)];
 x5=[x(5), x_hat(5)];
 x6=[x(6), x_hat(6)];
 x7=[x(7), x_hat(7)];
 x8=[x(8), x_hat(8)];
 x9=[x(9), x_hat(9)];
 x10=[x(10), x_hat(10)];
 x11=[x(11), x_hat(11)];
 x12=[x(12), x_hat(12)];

== matlab function main_simulation/Question 4/MATLAB Function1 ==
  data: u input size=4; xin input size=12; yout output size=4; x_dot output size=12
function [yout, x_dot] = fcn(u, xin)

L = 0.235; % m
Ix = 8.11858 * 10^(-5); % kg m2
Iy = 8.11858 * 10^(-5); % kg m2
Iz = 6.12233 * 10^(-5); % kg m2
b1 = L / Ix;
b2 = L / Iy;
b3 = L / Iz;
m = 0.506; % kg
g = 9.8; % m/s^2
a1 = (Iy - Iz) / Ix;
a2 = (Iz - Ix) / Iy;
a3 = (Ix - Iy) / Iz;

% Extracting values from xin
phi = xin(1);
phid = xin(2);
teta = xin(3);
tetad = xin(4);
psi = xin(5);
psid = xin(6);
z = xin(7);
zd = xin(8);
x = xin(9);
xd = xin(10);
y = xin(11);
yd = xin(12);

% Control input components
ut = cos(phi) * cos(teta);
ux = cos(phi) * sin(teta) * cos(psi) + sin(phi) * sin(psi);
uy = cos(phi) * sin(teta) * sin(psi) - sin(phi) * cos(psi);

% Output vector
yout = [phi; teta; psi; z];

% State derivatives
x_dot = [phid;
    tetad * psid * a1 + b1 * u(2);
    tetad;
    phid * psid * a2 + b2 * u(3);
    psid;
    phid * tetad * a3 + b3 * u(4);
    zd;
    -g + ut * (1 / m) * u(1);
    xd;
    ux * (1 / m) * u(1);
    yd;
    uy * (1 / m) * u(1)];
end

== matlab function main_simulation/part 1/Linear Model/MATLAB Function ==
  data: u input; y output; X input; x_dot output; A parameter; B parameter; C parameter
function [y,x_dot] = fcn(u, X, A, B, C)
    x_dot = A*X + B*u;
    y = C*X;

== matlab function main_simulation/part 1/Nonlinear Model/MATLAB Function ==
  data: U input; y output; X input; X_dot output; g parameter; m parameter; a1 parameter; a2 parameter; a3 parameter; b1 parameter; b2 parameter; b3 parameter; C parameter
function [y,X_dot] = fcn(U, X, g, m, a1, a2, a3, b1, b2, b3, C)
    X_dot = [X(2);
            X(4)*X(6)*a1 + b1*U(2);
            X(4);
            X(2)*X(6)*a2 + b2*U(3);
            X(6);
            X(2)*X(4)*a3+b3*U(4);
            X(8);
            -g + cos(X(1)) * cos(X(3)) * (1/m) * U(1);
            X(10);
            (cos(X(1))*sin(X(3))*cos(X(5)) - sin(X(1))*sin(X(5))) * (1/m) * U(1);
            X(12);
            (cos(X(1))*sin(X(3))*sin(X(5)) - sin(X(1))*cos(X(5))) * (1/m) * U(1)];
    y = C*X;

== matlab function main_simulation/part 3/states ==
  data: x input; x1 output; x_hat input; x2 output; x3 output; x4 output; x5 output; x6 output; x7 output; x8 output; x9 output; x10 output; x11 output; x12 output
function [x1 ,x2, x3, x4, x5, x6, x7, x8, x9, x10, x11, x12]  = CP(x, x_hat)

 x1=[x(1), x_hat(1)];
 x2=[x(2), x_hat(2)];
 x3=[x(3), x_hat(3)];
 x4=[x(4), x_hat(4)];
 x5=[x(5), x_hat(5)];
 x6=[x(6), x_hat(6)];
 x7=[x(7), x_hat(7)];
 x8=[x(8), x_hat(8)];
 x9=[x(9), x_hat(9)];
 x10=[x(10), x_hat(10)];
 x11=[x(11), x_hat(11)];
 x12=[x(12), x_hat(12)];

== matlab function main_simulation/part 3/MATLAB Function ==
  data: input input; y input; y1 output; y_hat input; y2 output; y3 output; y4 output
function [y1 ,y2 ,y3 ,y4]  = CP(input, y, y_hat)

 y1=[input(1), y(1), y_hat(1)];
 y2=[input(2), y(2), y_hat(2)];
 y3=[input(3), y(3), y_hat(3)];
 y4=[input(4), y(4), y_hat(4)];

== matlab function main_simulation/part 3/MATLAB Function1 ==
  data: input input; y input; y1 output; y_hat input; y2 output; y3 output; y4 output
function [y1 ,y2 ,y3 ,y4]  = CP(input, y, y_hat)

 y1=[input(1), y(1), y_hat(1)];
 y2=[input(2), y(2), y_hat(2)];
 y3=[input(3), y(3), y_hat(3)];
 y4=[input(4), y(4), y_hat(4)];

== matlab function main_simulation/part 3/states1 ==
  data: x input; x1 output; x_hat input; x2 output; x3 output; x4 output; x5 output; x6 output; x7 output; x8 output; x9 output; x10 output; x11 output; x12 output
function [x1 ,x2, x3, x4, x5, x6, x7, x8, x9, x10, x11, x12]  = CP(x, x_hat)

 x1=[x(1), x_hat(1)];
 x2=[x(2), x_hat(2)];
 x3=[x(3), x_hat(3)];
 x4=[x(4), x_hat(4)];
 x5=[x(5), x_hat(5)];
 x6=[x(6), x_hat(6)];
 x7=[x(7), x_hat(7)];
 x8=[x(8), x_hat(8)];
 x9=[x(9), x_hat(9)];
 x10=[x(10), x_hat(10)];
 x11=[x(11), x_hat(11)];
 x12=[x(12), x_hat(12)];

== matlab function main_simulation/part 3/MATLAB Function2 ==
  data: input input; y input; y1 output; y_hat input; y2 output; y3 output; y4 output
function [y1 ,y2 ,y3 ,y4]  = CP(input, y, y_hat)

 y1=[input(1), y(1), y_hat(1)];
 y2=[input(2), y(2), y_hat(2)];
 y3=[input(3), y(3), y_hat(3)];
 y4=[input(4), y(4), y_hat(4)];

== matlab function main_simulation/part 3/states2 ==
  data: x input; x1 output; x_hat input; x2 output; x3 output; x4 output; x5 output; x6 output; x7 output; x8 output; x9 output; x10 output; x11 output; x12 output
function [x1 ,x2, x3, x4, x5, x6, x7, x8, x9, x10, x11, x12]  = CP(x, x_hat)

 x1=[x(1), x_hat(1)];
 x2=[x(2), x_hat(2)];
 x3=[x(3), x_hat(3)];
 x4=[x(4), x_hat(4)];
 x5=[x(5), x_hat(5)];
 x6=[x(6), x_hat(6)];
 x7=[x(7), x_hat(7)];
 x8=[x(8), x_hat(8)];
 x9=[x(9), x_hat(9)];
 x10=[x(10), x_hat(10)];
 x11=[x(11), x_hat(11)];
 x12=[x(12), x_hat(12)];
